simulink model "Vejlupek_CAR4_dsPIC33_ACU44_SPI_R01"  (Simulink 7.3)
settings: Solver=FixedStepDiscrete  StartTime=0.0  StopTime=10.0  FixedStep=0.01  RelTol=1e-3
undefined symbols (not defined in the file or in its folder): PWM, QEIInit
libraries: dsPICdrivers x23, simulink x6
settings Model: Creator=Lubin  LastModifiedBy=Bobes
settings OptimizationCC: InlineParams=on  InlineInvariantSignals=on  InitFltsAndDblsToZero=on  OptimizeModelRefInitCode=on  LifeSpan=1
settings DebuggingCC: SaveWithParameterizedLinksMsg=none  SignalResolutionControl=TryResolveAllWithWarning
settings HardwareCC: ProdBitPerInt=16  ProdEndianess=LittleEndian  ProdWordSize=16  ProdHWDeviceType=16-bit Generic  TargetHWDeviceType=32-bit Generic
settings RTWCC: SystemTargetFile=dspic.tlc  TemplateMakefile=dspic_pic30_gcc.tmf  PostCodeGenCommand=dsPIC_Compile()  Description=Embedded Target for Microchip dsPIC (real-time)  GenerateReport=on  ProcessScript=dspic_make_rtw_hook  CustomSource=QEI_Functions.c  IncludeHyperlinkInReport=on  LaunchReport=on  GenerateTraceInfo=on  GenerateTraceReport=on  GenerateTraceReportSl=on  GenerateTraceReportSf=on  GenerateTraceReportEml=on
settings CodeAppCC: IgnoreCustomStorageClasses=off
settings STFCustomTargetCC: ModelReferenceCompliant=off  IncludeMdlTerminateFcn=off  CombineOutputUpdateFcns=on  SuppressErrorStatus=on  ERTCustomFileBanners=on  SupportContinuousTime=off  SupportNonInlinedSFcns=off  SystemTargetFile=dspic.tlc
settings ERTTargetCC: MultiwordLength=2048  ModelReferenceCompliant=off  ParMdlRefBuildCompliant=off  CompOptLevelCompliant=off  IncludeMdlTerminateFcn=off  SuppressErrorStatus=on  ERTFirstTimeCompliant=off  ModelStepFunctionPrototypeControlCompliant=off  CPPClassGenCompliant=off  InlinedParameterPlacement=NonHierarchical  ERTSrcFileBannerTemplate=dsPIC_code_template.cgt  ERTHdrFileBannerTemplate=dsPIC_code_template.cgt  ERTDataSrcFileTemplate=dsPIC_code_template.cgt  ERTDataHdrFileTemplate=dsPIC_code_template.cgt  ERTCustomFileTemplate=dsPIC_main.tlc
settings CustomProperty: DataType=string  Value=C:\PROGRA~1\MATLAB\R2009a\bin\win32\gmake

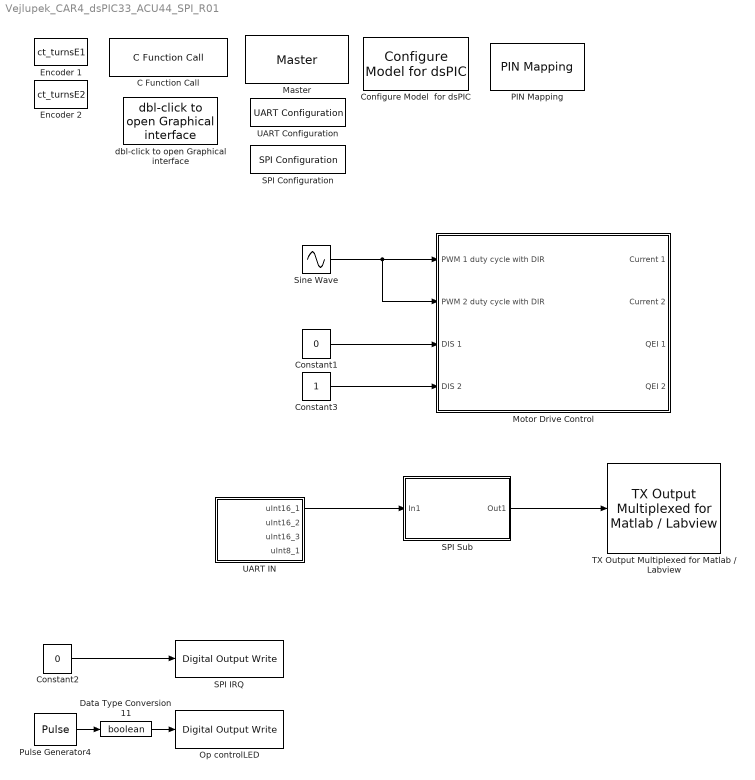
== system Vejlupek_CAR4_dsPIC33_ACU44_SPI_R01 ==
  C Function Call : dsPICdrivers/OTHERS/C Function Call  Tag=dsPIC_dsPIC_CFunctionCall  fctName='QEIInit'  INPUT_SIZE=1  INPUT1=--  INPUT2=--  INPUT3=--  OUTPUT_SIZE=1  OUTPUT1=--  SampleTime=inf  InputType=[ ]  OutputType=[ ]  FctDeclaration=extern void QEIInit();  FctCall=QEIInit();  OrderingInOutPopup=None
  Configure Model  for dsPIC : dsPICdrivers/Simulink Configuration/Configure Model  for dsPIC
  Constant1 : Constant  Value=0  OutDataTypeMode=boolean  OutDataType=fixdt(1, 16)  OutScaling=2^0  OutDataTypeStr=boolean  SampleTime=0.01
  Constant2 : Constant  Value=0  OutDataTypeMode=boolean  OutDataType=fixdt(1, 16)  OutScaling=2^0  OutDataTypeStr=boolean  SampleTime=0.01
  Constant3 : Constant  OutDataTypeMode=boolean  OutDataType=fixdt(1, 16)  OutScaling=2^0  OutDataTypeStr=boolean  SampleTime=0.01
  Data Type Conversion11 : DataTypeConversion  OutDataTypeMode=boolean  OutDataType=fixdt(1, 16)  OutScaling=2^0  OutDataTypeStr=boolean
  Encoder 1 : DataStoreMemory  DataStoreName=ct_turnsE1  ReadBeforeWriteMsg=warning  WriteAfterWriteMsg=warning  WriteAfterReadMsg=warning  DataType=uint16  OutDataType=sfix(16)  OutScaling=2^0  OutDataTypeStr=uint16
      settings: RTWStateStorageClass=ExportedGlobal
  Encoder 2 : DataStoreMemory  DataStoreName=ct_turnsE2  ReadBeforeWriteMsg=warning  WriteAfterWriteMsg=warning  WriteAfterReadMsg=warning  DataType=uint16  OutDataType=sfix(16)  OutScaling=2^0  OutDataTypeStr=uint16
      settings: RTWStateStorageClass=ExportedGlobal
  Master : dsPICdrivers/Master  Tag=dsPIC_MASTER  Priority=1  TimeStepType=Timer1  picType=33fj128MC804  fcy=20000000  Quartz_33f=20e6  PLLActive_33f=on  fcyDesired_33f=20000000  tmr1="[8  24999  0]"  tmr1Info="Time Step : 0.01  ;   Error : 0%  PR1=24999"  tmr2345="[0  0  0  0]"  tmr2345cfg=[-1 -1 -1 -1]  IOautoConf=on  typePort="[ 8   8   0   0   0   0   0  10  10   0  10   0   0   0   0   0   0   0  22  22  23   0   0  23  22  10  10   0   0   0   0   0  22  22  22  23   0   0  10   0   0  10   0   0   0   0   0   0   0   0   0   0   0   0   0   0   0   0   0   0   0   0   0   0   0   0   0   0   0   0   0   0   0   0   0   0   0   0   0   0   0   0   0   0   0   0   0   0   0   0   0   0   0   0   0   0   0   0   0   0   0   0   0   0   0   0   0   0   0   0   0   0 ]"  TRIS="[ 64127  63855  64951  65535  65535  65535  65535 ]"  ADPCFG=496  MasterBusyPort=None  MasterOverloadPort=None  FOSC=Quartz (XT - HS)  ClockSwitchMonitor=Both disabled  TempProtection_33f=TEMP_ON  FPBOR=<empty>  PWRT=64ms  MCLR=<empty>  PowerSave=off  OverrideFcy=off  NewFcy=1e6  PR2345="[65535  65535  65535  65535]"
  Motor Drive Control : Subsystem
  Op controlLED : dsPICdrivers/Digital I//O/Digital Output Write  Tag=dsPIC_Digital_Output  Priority=5  PORT=A  Pin=[8]  Simultaneous=off  OrderingInOutPopup=None
  PIN Mapping : dsPICdrivers/Peripheral MAPPING/PIN Mapping  Tag=dsPIC_PIN_Mapping  in_INT1=Not tied (VSS)  in_INT2=Not tied (VSS)  in_T2CK=Not tied (VSS)  in_T3CK=Not tied (VSS)  in_T4CK=Not tied (VSS)  in_T5CK=Not tied (VSS)  in_IC1=Not tied (VSS)  in_IC2=Not tied (VSS)  in_IC7=Not tied (VSS)  in_IC8=Not tied (VSS)  out_OC1=Not changed  out_OC2=Not changed  out_OC3=Not changed  out_OC4=Not changed  in_OCFA=Not tied (VSS)  in_FLTA1=Not tied (VSS)  in_FLTA2=Not tied (VSS)  in_QEA1=tied to RP16  in_QEB1=tied to RP17  in_INDX1=Not tied (VSS)  out_UPDN1=Not changed  out_UPDN2=Not changed  in_QEA2=tied to RP2  in_QEB2=tied to RP3  in_INDX2=Not tied (VSS)  in_U1RX=tied to RP18  out_U1TX=tied to RP4  in_U1CTS=Not tied (VSS)  out_U1RTS=Not changed  in_U2RX=Not changed  out_U2TX=Not changed  in_U2CTS=Not tied (VSS)  out_U2RTS=Not changed  in_SDI1=tied to RP8  out_SDO1=tied to RP19  in_SCK1=Not tied (VSS)  out_SCK1OUT=tied to RP7  in_SS1=Not tied (VSS)  out_SS1OUT=Not changed  in_SDI2=Not tied (VSS)  out_SDO2=Not changed  in_SCK2=Not tied (VSS)  out_SCK2OUT=Not changed  in_SS2=Not tied (VSS)  out_SS2OUT=Not changed  in_C1RX=Not tied (VSS)  out_C1TX=Not changed  out_C1OUT=Not changed  out_C2OUT=Not changed
  Pulse Generator4 : DiscretePulseGenerator  Amplitude=1  Period=100  PulseWidth=50  PhaseDelay=0  SampleTime=0.01
  SPI Configuration : dsPICdrivers/SPI PORT/SPI Configuration  Tag=dsPIC_config_SPI  Priority=2  ConfigurationTime=At boot time (only once)  OrderingInOutPopup=None  SampleTime=-1  Frame_Enable=0  Frame_Sync=None  SPI=1  MODE=MASTER  USER_SCALER=96  StartEnable=Enable  SDO_EN=off  DATA_LENGTH=16 bits  SS_EN=off  SMP=End of bit  CKP=high  CKE=Idle to Active  Status="OK - Mode 1  -    Fsck= 208333.3333Hz"
  SPI IRQ : dsPICdrivers/Digital I//O/Digital Output Write  Tag=dsPIC_Digital_Output  Priority=5  PORT=C  Pin=[6]  Simultaneous=off  OrderingInOutPopup=None
  SPI Sub : Subsystem  TreatAsAtomicUnit=on
  Sine Wave : Sin  SineType=Sample based  Amplitude=PWM*0.9  Bias=0  Frequency=1  Phase=0  Samples=10e2  SampleTime=1e-2  Offset=0
  TX Output Multiplexed for Matlab / Labview : dsPICdrivers/Serial PORT/TX Output Multiplexed for Matlab // Labview  Tag=dsPIC_TX_Multiplexed  Priority=5  UART=1  CleverSpreadingChk=on  CleverSpreading=1  CHANNEL=[0]  CHANNELBLOCKED=[]  CHANNELBLOCKED_BITEWISE=0  Status=OK
  UART Configuration : dsPICdrivers/Serial PORT/UART Configuration  Tag=dsPIC_config_UART  Priority=2  UART=1  proposed_BAUD=9600  ALT_TX_RX=on  InterruptTxWhen=When Transmit Buffer is empty  TXInterruptPri=1  TxBufferSize=32  TXEN=on  InterruptRxWhen=When Receive Buffer is full (contain 4 characters)  RXInterruptPri=2  RxBufferSize=32  BAUD=9600  UxBRG=129  Info="UxBRG = 129   ||  Real Baud : 9615   ||  % error : 0.16026  ||  max 9.6154 Bytes / Step"  RealBaud=0
  UART IN : Subsystem
  dbl-click to open Graphical interface : dsPICdrivers/Serial PORT/dbl-click to open Graphical interface  SystemSampleTime=-1  Nothing=0
  wires:
  Sine Wave/1 -> Motor Drive Control/1(PWM 1 duty cycle with DIR), Motor Drive Control/2(PWM 2 duty cycle with DIR)
  Data Type Conversion11/1 -> Op controlLED/1
  Pulse Generator4/1 -> Data Type Conversion11/1
  Constant1/1 -> Motor Drive Control/3(DIS 1)
  Constant3/1 -> Motor Drive Control/4(DIS 2)
  Constant2/1 -> SPI IRQ/1
  UART IN/1(uInt16_1) -> SPI Sub/1(In1)
  SPI Sub/1(Out1) -> TX Output Multiplexed for Matlab / Labview/1

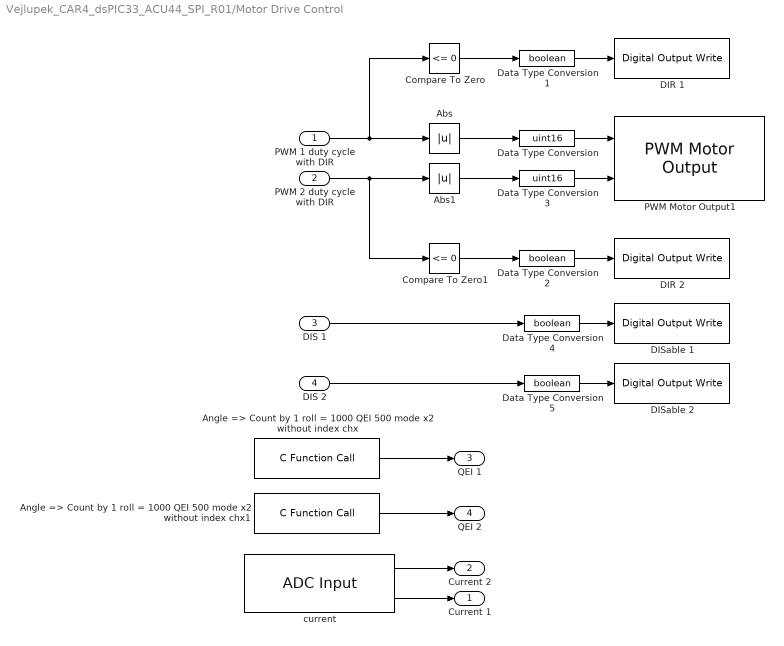
== system Vejlupek_CAR4_dsPIC33_ACU44_SPI_R01/Motor Drive Control ==
  PWM 1 duty cycle with DIR : Inport
  PWM 2 duty cycle with DIR : Inport  Port=2
  DIS 1 : Inport  Port=3
  DIS 2 : Inport  Port=4
  Abs : Abs  OutDataType=fixdt(1, 16)  OutScaling=2^0
  Abs1 : Abs  OutDataType=fixdt(1, 16)  OutScaling=2^0
  Angle => Count by 1 roll = 1000 QEI 500 mode x2 without index chx : dsPICdrivers/OTHERS/C Function Call  Tag=dsPIC_dsPIC_CFunctionCall  fctName='GetQEI1'  INPUT_SIZE=1  INPUT1=--  INPUT2=--  INPUT3=--  OUTPUT_SIZE=1  OUTPUT1=uint16  SampleTime=-1  InputType=[ ]  OutputType=[ 4 ]  FctDeclaration=extern uint16_T GetQEI1();  FctCall=%y1 = GetQEI1();  OrderingInOutPopup=None
  Angle => Count by 1 roll = 1000 QEI 500 mode x2 without index chx1 : dsPICdrivers/OTHERS/C Function Call  Tag=dsPIC_dsPIC_CFunctionCall  fctName='GetQEI2'  INPUT_SIZE=1  INPUT1=--  INPUT2=--  INPUT3=--  OUTPUT_SIZE=1  OUTPUT1=uint16  SampleTime=-1  InputType=[ ]  OutputType=[ 4 ]  FctDeclaration=extern uint16_T GetQEI2();  FctCall=%y1 = GetQEI2();  OrderingInOutPopup=None
  Compare To Zero : simulink/Logic and Bit Operations/Compare To Zero  SystemSampleTime=-1  relop=<=  LogicOutDataTypeMode=boolean  ZeroCross=off
  Compare To Zero1 : simulink/Logic and Bit Operations/Compare To Zero  SystemSampleTime=-1  relop=<=  LogicOutDataTypeMode=boolean  ZeroCross=off
  DIR 1 : dsPICdrivers/Digital I//O/Digital Output Write  Tag=dsPIC_Digital_Output  Priority=5  PORT=A  Pin=[10]  Simultaneous=off  OrderingInOutPopup=None
  DIR 2 : dsPICdrivers/Digital I//O/Digital Output Write  Tag=dsPIC_Digital_Output  Priority=5  PORT=B  Pin=[10]  Simultaneous=off  OrderingInOutPopup=None
  DISable 1 : dsPICdrivers/Digital I//O/Digital Output Write  Tag=dsPIC_Digital_Output  Priority=5  PORT=A  Pin=[7]  Simultaneous=off  OrderingInOutPopup=None
  DISable 2 : dsPICdrivers/Digital I//O/Digital Output Write  Tag=dsPIC_Digital_Output  Priority=5  PORT=C  Pin=[9]  Simultaneous=off  OrderingInOutPopup=None
  Data Type Conversion : DataTypeConversion  OutDataTypeMode=uint16  OutDataType=fixdt(1, 16)  OutScaling=2^0  OutDataTypeStr=uint16
  Data Type Conversion{1..2,4..5} (4 alike) : DataTypeConversion  OutDataTypeMode=boolean  OutDataType=fixdt(1, 16)  OutScaling=2^0  OutDataTypeStr=boolean
  Data Type Conversion3 : DataTypeConversion  OutDataTypeMode=uint16  OutDataType=fixdt(1, 16)  OutScaling=2^0  OutDataTypeStr=uint16
  PWM Motor Output1 : dsPICdrivers/Peripheral I//O/PWM Motor Output  Tag=dsPIC_PWM_Motor  Priority=5  PWMref=1  PWM12=2  InputEnableChk=off  InputPeriodeChk=off  Channel=[1 2]  TPeriode=.0001  PrescalerValue=1  PeriodeInteger=2000  MaxName='PWM'  Centered=off  HChannelON=off  Info="Nbr Bits : 11.9658  ||  PWM = 4000  ||  Prescaler = 1"  Delay=0  IntPriority=5  nbrPwmChannelPIC=3  Status=OK  DeadTimePrescaleA=0  DeadTimePrescaleB=0  DeadTimeInfo="Dead Time A = 0  ||  Dead Time B = 0"  DTPWM1a=Prescaler A  DTPWM1i=Prescaler A  DTPWM2a=Prescaler A  DTPWM2i=Prescaler A  DTPWM3a=Prescaler A  DTPWM3i=Prescaler A  DTPWM4a=Prescaler A  DTPWM4i=Prescaler A  DTCON1=0  DTCON2=0
  current : dsPICdrivers/Peripheral I//O/ADC Input  Tag=dsPIC_ADC  Priority=5  ADC_TYPE=12 bits  ADC_MODE=Continuous sampling & get last channel value  NbrSampleStep=1  VoltRefpopup="AVdd  -  AVss"  OutFormatBitspopup=0000 dddd dddd dddd : Integer  InterruptPriority=6  ANCHANNELS=[0 1]  MaxName=ANmax = 4095  Rin=1e2  ADCS=26  SAMC=1  Temperature=25  DMAChannel=0  SampleTime=0.01  Status="OK  |  Tsmp=6.750e-007 |  T/Channel=1.012e-005 |  Tall=2.025e-005"  SSRC=auto convert
  Current 1 : Outport
  Current 2 : Outport  Port=2
  QEI 1 : Outport  Port=3
  QEI 2 : Outport  Port=4
  wires:
  Data Type Conversion1/1 -> DIR 1/1
  Data Type Conversion/1 -> PWM Motor Output1/1
  Compare To Zero/1 -> Data Type Conversion1/1
  PWM 1 duty cycle with DIR/1 -> Compare To Zero/1, Abs/1
  Abs/1 -> Data Type Conversion/1
  Angle => Count by 1 roll = 1000 QEI 500 mode x2 without index chx1/1 -> QEI 2/1
  Angle => Count by 1 roll = 1000 QEI 500 mode x2 without index chx/1 -> QEI 1/1
  PWM 2 duty cycle with DIR/1 -> Abs1/1, Compare To Zero1/1
  Abs1/1 -> Data Type Conversion3/1
  Compare To Zero1/1 -> Data Type Conversion2/1
  Data Type Conversion2/1 -> DIR 2/1
  Data Type Conversion3/1 -> PWM Motor Output1/2
  DIS 1/1 -> Data Type Conversion4/1
  DIS 2/1 -> Data Type Conversion5/1
  Data Type Conversion4/1 -> DISable 1/1
  Data Type Conversion5/1 -> DISable 2/1
  current/1 -> Current 2/1
  current/2 -> Current 1/1

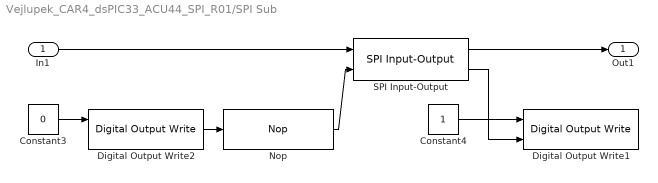
== system Vejlupek_CAR4_dsPIC33_ACU44_SPI_R01/SPI Sub ==
  In1 : Inport
  Constant3 : Constant  Value=0  OutDataTypeMode=boolean  OutDataType=sfix(16)  OutScaling=2^0  OutDataTypeStr=boolean
  Constant4 : Constant  OutDataTypeMode=boolean  OutDataType=sfix(16)  OutScaling=2^0  OutDataTypeStr=boolean
  Digital Output Write1 : dsPICdrivers/Digital I//O/Digital Output Write  Tag=dsPIC_Digital_Output  Priority=5  PORT=B  Pin=[9]  Simultaneous=off  OrderingInOutPopup=Input
  Digital Output Write2 : dsPICdrivers/Digital I//O/Digital Output Write  Tag=dsPIC_Digital_Output  Priority=5  PORT=B  Pin=[9]  Simultaneous=off  OrderingInOutPopup=Input & Output
  Nop : dsPICdrivers/OTHERS/Nop  Tag=dsPIC_Reset  NbrNop=5
  SPI Input-Output : dsPICdrivers/SPI PORT/SPI Input-Output  Tag=dsPIC_SPI  SPI=1  INPUT=on  RESET_INPUT=on  OUTPUT=on  SPECIAL_SPI=Always Enable  DATA_LENGTH=16 bits  WAIT_INPUTDATA=on  OrderingInOutPopup=Input & Output  SampleTime=-1
  Out1 : Outport
  wires:
  In1/1 -> SPI Input-Output/1
  SPI Input-Output/1 -> Out1/1
  Constant3/1 -> Digital Output Write2/1
  Digital Output Write2/1 -> Nop/1
  SPI Input-Output/2 -> Digital Output Write1/2
  Constant4/1 -> Digital Output Write1/1
  Nop/1 -> SPI Input-Output/2

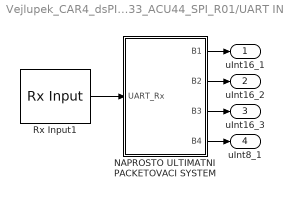
== system Vejlupek_CAR4_dsPIC33_ACU44_SPI_R01/UART IN ==
  NAPROSTO ULTIMATNI PACKETOVACI SYSTEM : Subsystem
  Rx Input1 : dsPICdrivers/Serial PORT/Rx Input  Tag=dsPIC_RX  Priority=5  UART=1  SampleTime=0.01  BlockingFctChk=off  OutputDefault=0  IsPresentFlagChk=off
  uInt16_1 : Outport
  uInt16_2 : Outport  Port=2
  uInt16_3 : Outport  Port=3
  uInt8_1 : Outport  Port=4
  wires:
  Rx Input1/1 -> NAPROSTO ULTIMATNI PACKETOVACI SYSTEM/1(UART_Rx)
  NAPROSTO ULTIMATNI PACKETOVACI SYSTEM/1(B1) -> uInt16_1/1
  NAPROSTO ULTIMATNI PACKETOVACI SYSTEM/2(B2) -> uInt16_2/1
  NAPROSTO ULTIMATNI PACKETOVACI SYSTEM/3(B3) -> uInt16_3/1
  NAPROSTO ULTIMATNI PACKETOVACI SYSTEM/4(B4) -> uInt8_1/1

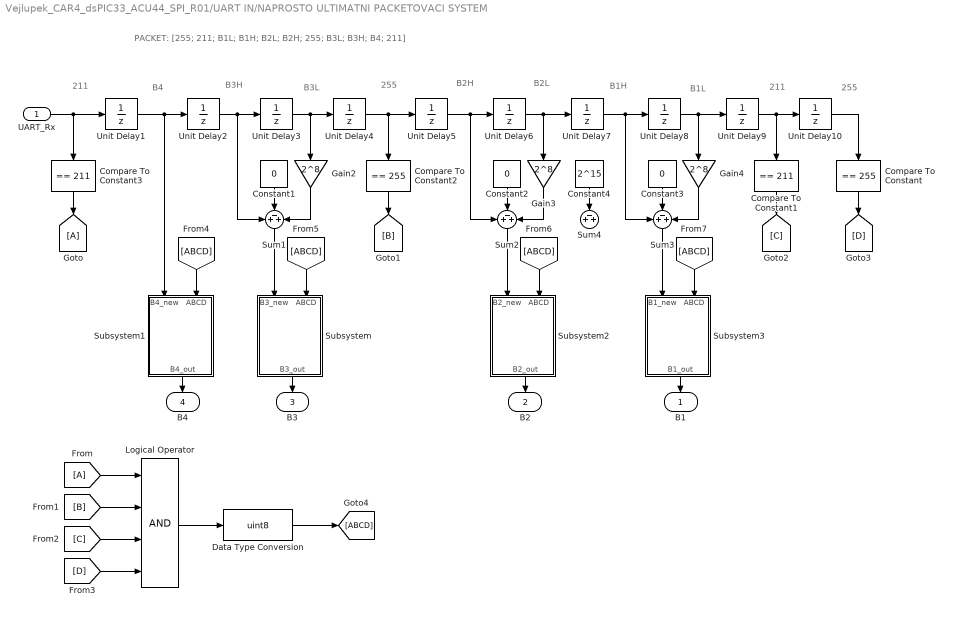
== system Vejlupek_CAR4_dsPIC33_ACU44_SPI_R01/UART IN/NAPROSTO ULTIMATNI PACKETOVACI SYSTEM ==
  note: PACKET: [255; 211; B1L; B1H; B2L; B2H; 255; B3L; B3H; B4; 211]
  note: 211
  note: B4
  note: B3H
  note: B3L
  note: 255
  note: B2H
  note: B2L
  note: B1H
  note: B1L
  note: 211
  note: 255
  UART_Rx : Inport
  Compare To Constant : simulink/Logic and Bit Operations/Compare To Constant  SystemSampleTime=-1  relop===  const=255  LogicOutDataTypeMode=boolean  ZeroCross=off
  Compare To Constant1 : simulink/Logic and Bit Operations/Compare To Constant  SystemSampleTime=-1  relop===  const=211  LogicOutDataTypeMode=boolean  ZeroCross=off
  Compare To Constant2 : simulink/Logic and Bit Operations/Compare To Constant  SystemSampleTime=-1  relop===  const=255  LogicOutDataTypeMode=boolean  ZeroCross=off
  Compare To Constant3 : simulink/Logic and Bit Operations/Compare To Constant  SystemSampleTime=-1  relop===  const=211  LogicOutDataTypeMode=boolean  ZeroCross=off
  Constant1 : Constant  Value=0  OutDataTypeMode=uint16  OutDataType=fixdt(1, 16)  OutScaling=2^0  OutDataTypeStr=uint16
  Constant2 : Constant  Value=0  OutDataTypeMode=uint16  OutDataType=fixdt(1, 16)  OutScaling=2^0  OutDataTypeStr=uint16
  Constant3 : Constant  Value=0  OutDataTypeMode=uint16  OutDataType=fixdt(1, 16)  OutScaling=2^0  OutDataTypeStr=uint16
  Constant4 : Constant  Value=2^15  OutDataTypeMode=uint16  OutDataType=fixdt(1, 16)  OutScaling=2^0  OutDataTypeStr=uint16
  Data Type Conversion : DataTypeConversion  OutDataTypeMode=uint8  OutDataType=fixdt(1, 16)  OutScaling=2^0  OutDataTypeStr=uint8
  Gain2 : Gain  Gain=2^8  ParameterDataType=fixdt(1, 16)  ParameterScaling=2^0  OutDataTypeMode=uint16  OutDataType=fixdt(1, 16)  OutScaling=2^0  OutDataTypeStr=uint16
  Gain3 : Gain  Gain=2^8  ParameterDataType=fixdt(1, 16)  ParameterScaling=2^0  OutDataTypeMode=uint16  OutDataType=fixdt(1, 16)  OutScaling=2^0  OutDataTypeStr=uint16
  Gain4 : Gain  Gain=2^8  ParameterDataType=fixdt(1, 16)  ParameterScaling=2^0  OutDataTypeMode=uint16  OutDataType=fixdt(1, 16)  OutScaling=2^0  OutDataTypeStr=uint16
  Logical Operator : Logic  Inputs=4  AllPortsSameDT=off  OutDataTypeMode=boolean  LogicDataType=fixdt(0, 8)  OutDataTypeStr=boolean
  Subsystem : Subsystem
  Subsystem1 : Subsystem
  Subsystem2 : Subsystem
  Subsystem3 : Subsystem
  Sum1 : Sum  Inputs=+-+  AccumDataTypeStr=int32  OutDataTypeMode=uint16  OutDataType=fixdt(1, 16)  OutScaling=2^0  OutDataTypeStr=uint16
  Sum2 : Sum  Inputs=+-+  AccumDataTypeStr=int32  OutDataTypeMode=uint16  OutDataType=fixdt(1, 16)  OutScaling=2^0  OutDataTypeStr=uint16
  Sum3 : Sum  Inputs=+-+  AccumDataTypeStr=int32  OutDataTypeMode=uint16  OutDataType=fixdt(1, 16)  OutScaling=2^0  OutDataTypeStr=uint16
  Sum4 : Sum  Inputs=+-+  AccumDataTypeStr=int32  OutDataTypeMode=int16  OutDataType=fixdt(1, 16)  OutScaling=2^0  OutDataTypeStr=int16
  Unit Delay{1..10} (10 alike) : UnitDelay  SampleTime=-1
  B1 : Outport  OutDataType=fixdt(1, 16)  OutScaling=2^0
  B2 : Outport  Port=2  OutDataType=fixdt(1, 16)  OutScaling=2^0
  B3 : Outport  Port=3  OutDataType=fixdt(1, 16)  OutScaling=2^0
  B4 : Outport  Port=4  OutDataType=fixdt(1, 16)  OutScaling=2^0
  wires:
  UART_Rx/1 -> Unit Delay1/1, Compare To Constant3/1
  Unit Delay1/1 -> Unit Delay2/1, Subsystem1/1(B4_new)
  Unit Delay2/1 -> Unit Delay3/1, Sum1/1
  Unit Delay3/1 -> Unit Delay4/1, Gain2/1
  Unit Delay4/1 -> Unit Delay5/1, Compare To Constant2/1
  Unit Delay5/1 -> Unit Delay6/1, Sum2/1
  Unit Delay6/1 -> Unit Delay7/1, Gain3/1
  Unit Delay7/1 -> Unit Delay8/1, Sum3/1
  Unit Delay8/1 -> Unit Delay9/1, Gain4/1
  Unit Delay9/1 -> Unit Delay10/1, Compare To Constant1/1
  Unit Delay10/1 -> Compare To Constant/1
  Constant1/1 -> Sum1/2
  Gain2/1 -> Sum1/3
  Constant2/1 -> Sum2/2
  Gain3/1 -> Sum2/3
  Constant3/1 -> Sum3/2
  Gain4/1 -> Sum3/3
  Compare To Constant3/1 -> [A]
  Compare To Constant2/1 -> [B]
  Compare To Constant1/1 -> [C]
  Compare To Constant/1 -> [D]
  [A] -> Logical Operator/1
  [B] -> Logical Operator/2
  [C] -> Logical Operator/3
  [D] -> Logical Operator/4
  Logical Operator/1 -> Data Type Conversion/1
  Data Type Conversion/1 -> [ABCD]
  Sum1/1 -> Subsystem/1(B3_new)
  Subsystem/1(B3_out) -> B3/1
  Subsystem1/1(B4_out) -> B4/1
  Subsystem2/1(B2_out) -> B2/1
  Subsystem3/1(B1_out) -> B1/1
  Sum3/1 -> Subsystem3/1(B1_new)
  Sum2/1 -> Subsystem2/1(B2_new)
  [ABCD] -> Subsystem1/2(ABCD)
  [ABCD] -> Subsystem3/2(ABCD)
  [ABCD] -> Subsystem2/2(ABCD)
  [ABCD] -> Subsystem/2(ABCD)
  Constant4/1 -> Sum4/2

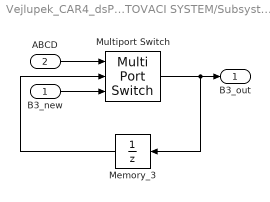
== system Vejlupek_CAR4_dsPIC33_ACU44_SPI_R01/UART IN/NAPROSTO ULTIMATNI PACKETOVACI SYSTEM/Subsystem ==
  B3_new : Inport
  ABCD : Inport  Port=2
  Memory_3 : UnitDelay  SampleTime=-1
  Multiport Switch : MultiPortSwitch  Inputs=2  zeroidx=on  OutDataTypeMode=uint16  OutDataType=fixdt(1, 16)  OutScaling=2^0  OutDataTypeStr=uint16
  B3_out : Outport
  wires:
  ABCD/1 -> Multiport Switch/1
  Multiport Switch/1 -> Memory_3/1, B3_out/1
  Memory_3/1 -> Multiport Switch/2
  B3_new/1 -> Multiport Switch/3

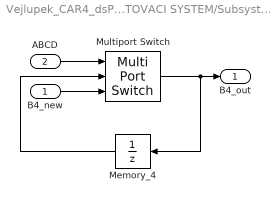
== system Vejlupek_CAR4_dsPIC33_ACU44_SPI_R01/UART IN/NAPROSTO ULTIMATNI PACKETOVACI SYSTEM/Subsystem1 ==
  B4_new : Inport
  ABCD : Inport  Port=2
  Memory_4 : UnitDelay  SampleTime=-1
  Multiport Switch : MultiPortSwitch  Inputs=2  zeroidx=on  OutDataTypeMode=uint8  OutDataType=fixdt(1, 16)  OutScaling=2^0  OutDataTypeStr=uint8
  B4_out : Outport
  wires:
  B4_new/1 -> Multiport Switch/3
  Memory_4/1 -> Multiport Switch/2
  Multiport Switch/1 -> B4_out/1, Memory_4/1
  ABCD/1 -> Multiport Switch/1

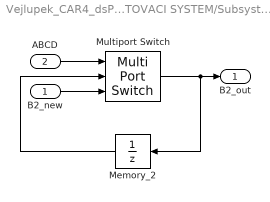
== system Vejlupek_CAR4_dsPIC33_ACU44_SPI_R01/UART IN/NAPROSTO ULTIMATNI PACKETOVACI SYSTEM/Subsystem2 ==
  B2_new : Inport
  ABCD : Inport  Port=2
  Memory_2 : UnitDelay  SampleTime=-1
  Multiport Switch : MultiPortSwitch  Inputs=2  zeroidx=on  OutDataTypeMode=uint16  OutDataType=fixdt(1, 16)  OutScaling=2^0  OutDataTypeStr=uint16
  B2_out : Outport
  wires:
  B2_new/1 -> Multiport Switch/3
  Memory_2/1 -> Multiport Switch/2
  Multiport Switch/1 -> B2_out/1, Memory_2/1
  ABCD/1 -> Multiport Switch/1

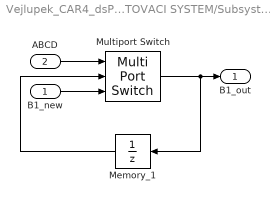
== system Vejlupek_CAR4_dsPIC33_ACU44_SPI_R01/UART IN/NAPROSTO ULTIMATNI PACKETOVACI SYSTEM/Subsystem3 ==
  B1_new : Inport
  ABCD : Inport  Port=2
  Memory_1 : UnitDelay  SampleTime=-1
  Multiport Switch : MultiPortSwitch  Inputs=2  zeroidx=on  OutDataTypeMode=uint16  OutDataType=fixdt(1, 16)  OutScaling=2^0  OutDataTypeStr=uint16
  B1_out : Outport
  wires:
  ABCD/1 -> Multiport Switch/1
  Multiport Switch/1 -> Memory_1/1, B1_out/1
  Memory_1/1 -> Multiport Switch/2
  B1_new/1 -> Multiport Switch/3
